simulink model "Controller_v2_testing"  (R2025b)
settings: Solver=VariableStepAuto  StartTime=0.0  StopTime=2  RelTol=1e-3
InitFcn:
  | q_upright = [cosd(45);0;sind(45);0];
  | 
  | q_roll10 = quatmultiply( ...
  |     [cosd(45) 0 sind(45) 0], ...
  |     [cosd(5) sind(5) 0 0]);
  | q_roll10 = [ 0.7044160;
  |                   -0.0616284;
  |                    0.7044160;
  |                    0.0616284];
settings Model: Creator=Admin  LastModifiedBy=Admin

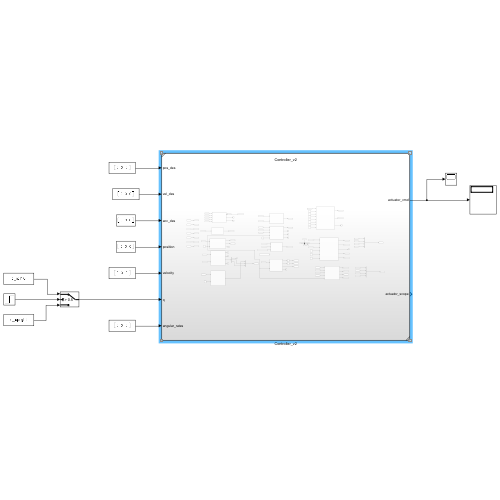
[thumbnail: Simulink's stored preview of the top-level diagram]
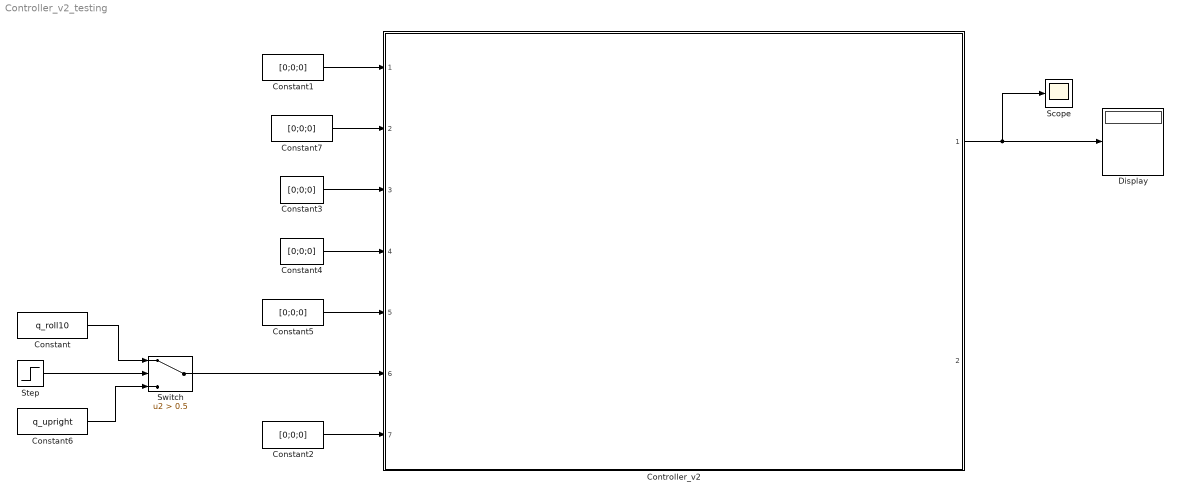
== system Controller_v2_testing ==
  Constant : Constant  Value=q_roll10
  Constant{1..5,7} (6 alike) : Constant  Value=[0;0;0]
  Constant6 : Constant  Value=q_upright
  Controller_v2 : Subsystem  ReferencedSubsystem=Controller_v2
  Display : Display
  Scope : Scope
      settings: ActiveDisplayYMinimum=58.059600683950585  ActiveDisplayYMaximum=59.219499730546119
  Step : Step  SampleTime=0
  Switch : Switch  Criteria=u2 > Threshold  Threshold=0.5  SaturateOnIntegerOverflow=off  InputSameDT=off
  wires:
  Controller_v2/1 -> Display/1, Scope/1
  Constant1/1 -> Controller_v2/1
  Constant7/1 -> Controller_v2/2
  Constant3/1 -> Controller_v2/3
  Constant4/1 -> Controller_v2/4
  Constant5/1 -> Controller_v2/5
  Constant2/1 -> Controller_v2/7
  Step/1 -> Switch/2
  Constant/1 -> Switch/1
  Constant6/1 -> Switch/3
  Switch/1 -> Controller_v2/6
